simulink model "ventilation_I"  (R2026a)
settings: Solver=FixedStepDiscrete  StopTime=60  FixedStep=Ts
model workspace (MAT data in the model file):
  Ts = 1
  r_set = 300
Description:
  | UESTCHN4002 Computer Lab 3, Exercise 3B: ventilation-rate control loop
settings Model: Creator=ChenKe  LastModifiedBy=alan

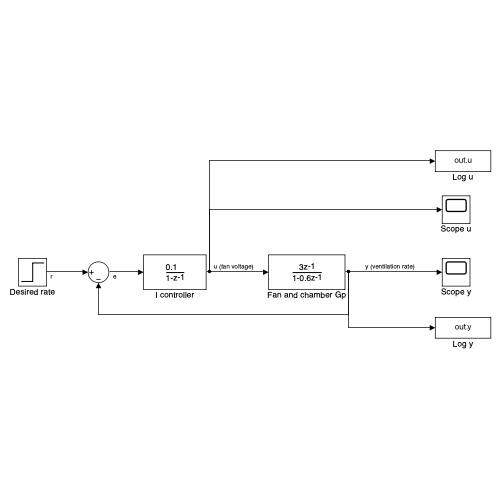
[thumbnail: Simulink's stored preview of the top-level diagram]
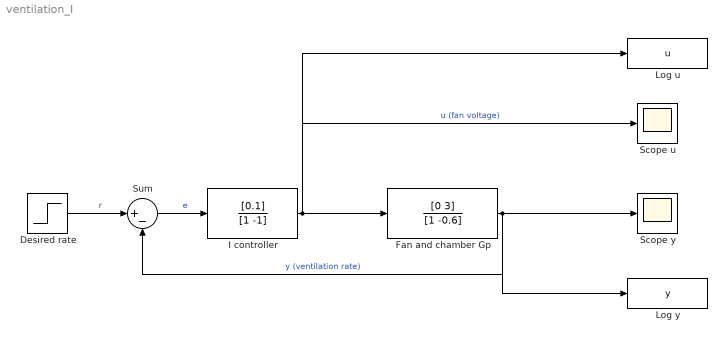
== system ventilation_I ==
  Desired rate : Step  Time=0  FinalValue=r_set  SampleTime=Ts
  Fan and chamber Gp : DiscreteFilter  Numerator=[0 3]  Denominator=[1 -0.6]  SampleTime=Ts
  I controller : DiscreteFilter  Numerator=[0.1]  Denominator=[1 -1]  SampleTime=Ts
  Log u : ToWorkspace  VariableName=u  SaveFormat=Timeseries  SampleTime=Ts
  Log y : ToWorkspace  VariableName=y  SaveFormat=Timeseries  SampleTime=Ts
  Scope u : Scope
  Scope y : Scope
  Sum : Sum  Inputs=|+-
  wires:
  Desired rate/1 -> Sum/1  "r"
  Sum/1 -> I controller/1  "e"
  I controller/1 -> Fan and chamber Gp/1, Scope u/1, Log u/1  "u (fan voltage)"
  Fan and chamber Gp/1 -> Scope y/1, Log y/1, Sum/2  "y (ventilation rate)"
